simulink model "inclass1006"  (R2026a)
settings: Solver=FixedStepAuto  StopTime=inf  FixedStep=0.05
libraries: robotlib x9
settings Model: Creator=sprinkle  LastModifiedBy=sprinkle
settings HardwareCC: ProdHWDeviceType=Generic->Unspecified (assume 32-bit Generic)
settings RTWCC: SystemTargetFile=ert.tlc  HardwareBoard=Robot Operating System (ROS)  TLCOptions="-aInlineSetEventsForThisBaseRateFcn=TLC_FALSE -aSuppressMultiTaskScheduler=TLC_FALSE  -aRateBasedStepFcn=0"  GenCodeOnly=on  Toolchain=Catkin  TargetLang=C++  Description=Embedded Coder

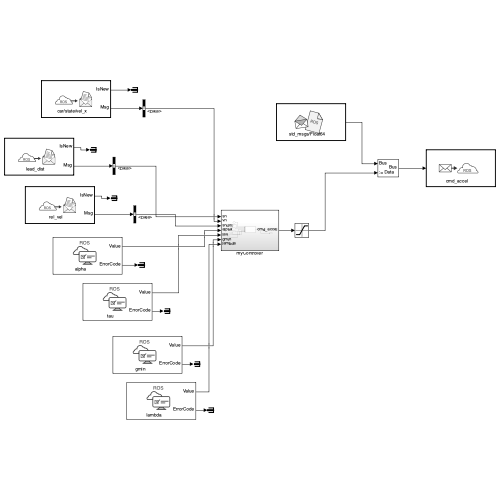
[thumbnail: Simulink's stored preview of the top-level diagram]
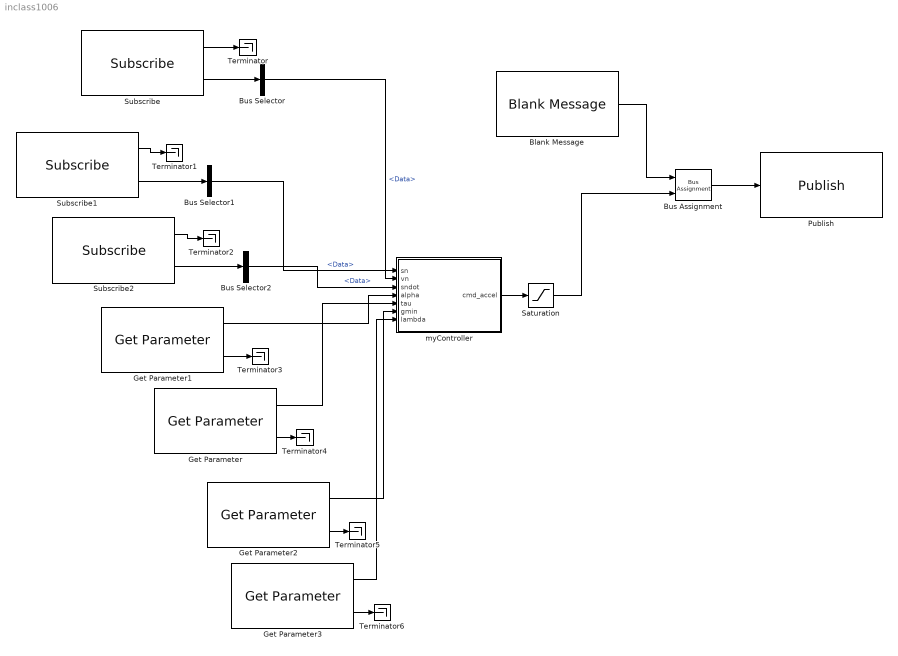
== system inclass1006 ==
  Blank Message : robotlib/Blank Message  messageClass=Message  entityType=std_msgs/Float64  messageType=std_msgs/Float64  SampleTime=inf  legacyBusStruct=off
  Bus Assignment : BusAssignment  AssignedSignals=Data
  Bus Selector : BusSelector  OutputSignals=Data
  Bus Selector1 : BusSelector  OutputSignals=Data
  Bus Selector2 : BusSelector  OutputSignals=Data
  Get Parameter : robotlib/Get Parameter  ParameterSource=Specify your own  ParameterName=tau  ParameterType=double  ParameterMaxArrayLength=16  ParameterInitialValue=2.0  SampleTime=-1  ShowErrorCodeOutput=on  ModelName=inclass1006  BlockId=ParamGet_inclass1006_18
  Get Parameter1 : robotlib/Get Parameter  ParameterSource=Specify your own  ParameterName=alpha  ParameterType=double  ParameterMaxArrayLength=16  ParameterInitialValue=1.1  SampleTime=-1  ShowErrorCodeOutput=on  ModelName=inclass1006  BlockId=ParamGet_inclass1006_19
  Get Parameter2 : robotlib/Get Parameter  ParameterSource=Specify your own  ParameterName=gmin  ParameterType=double  ParameterMaxArrayLength=16  ParameterInitialValue=3  SampleTime=-1  ShowErrorCodeOutput=on  ModelName=inclass1006  BlockId=ParamGet_inclass1006_52
  Get Parameter3 : robotlib/Get Parameter  ParameterSource=Specify your own  ParameterName=lambda  ParameterType=double  ParameterMaxArrayLength=16  ParameterInitialValue=0.1  SampleTime=-1  ShowErrorCodeOutput=on  ModelName=inclass1006  BlockId=ParamGet_inclass1006_52
  Publish : robotlib/Publish  topicSource=Specify your own  topic=cmd_accel  messageType=std_msgs/Float64  legacyBusStruct=off  messageQueueLength=1
  Saturation : Saturate  UpperLimit=1.5  LowerLimit=-3.0
  Subscribe : robotlib/Subscribe  topicSource=Specify your own  topic=car/state/vel_x  messageType=std_msgs/Float64  SampleTime=-1  legacyBusStruct=off  messageQueueLength=1
  Subscribe1 : robotlib/Subscribe  topicSource=Specify your own  topic=lead_dist  messageType=std_msgs/Float64  SampleTime=-1  legacyBusStruct=off  messageQueueLength=1
  Subscribe2 : robotlib/Subscribe  topicSource=Specify your own  topic=rel_vel  messageType=std_msgs/Float64  SampleTime=-1  legacyBusStruct=off  messageQueueLength=1
  Terminator{,1..6} (7 alike) : Terminator
  myController : Subsystem
  wires:
  Subscribe/2 -> Bus Selector/1
  Subscribe/1 -> Terminator/1
  Subscribe1/1 -> Terminator1/1
  Blank Message/1 -> Bus Assignment/1
  Bus Assignment/1 -> Publish/1
  Bus Selector/1 -> myController/2(vn)  "<Data>"
  myController/1(cmd_accel) -> Saturation/1
  Get Parameter/1 -> myController/5(tau)
  Get Parameter1/1 -> myController/4(alpha)
  Saturation/1 -> Bus Assignment/2
  Subscribe1/2 -> Bus Selector1/1
  Bus Selector1/1 -> myController/1(sn)  "<Data>"
  Subscribe2/1 -> Terminator2/1
  Bus Selector2/1 -> myController/3(sndot)  "<Data>"
  Subscribe2/2 -> Bus Selector2/1
  Get Parameter1/2 -> Terminator3/1
  Get Parameter/2 -> Terminator4/1
  Get Parameter2/2 -> Terminator5/1
  Get Parameter3/2 -> Terminator6/1
  Get Parameter2/1 -> myController/6(gmin)
  Get Parameter3/1 -> myController/7(lambda)

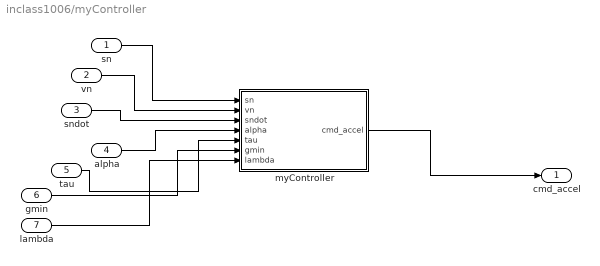
== system inclass1006/myController ==
  sn : Inport
  vn : Inport  Port=2
  sndot : Inport  Port=3
  alpha : Inport  Port=4
  tau : Inport  Port=5
  gmin : Inport  Port=6
  lambda : Inport  Port=7
  myController : Subsystem
  cmd_accel : Outport
  wires:
  myController/1(cmd_accel) -> cmd_accel/1
  tau/1 -> myController/5(tau)
  alpha/1 -> myController/4(alpha)
  sn/1 -> myController/1(sn)
  vn/1 -> myController/2(vn)
  sndot/1 -> myController/3(sndot)
  gmin/1 -> myController/6(gmin)
  lambda/1 -> myController/7(lambda)

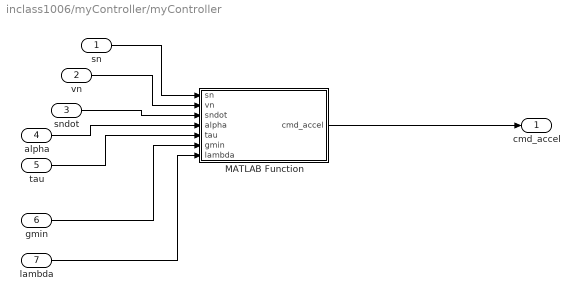
== system inclass1006/myController/myController ==
  sn : Inport
  vn : Inport  Port=2
  sndot : Inport  Port=3
  alpha : Inport  Port=4
  tau : Inport  Port=5
  gmin : Inport  Port=6
  lambda : Inport  Port=7
  MATLAB Function : MATLAB Function  TreatAsAtomicUnit=on
  cmd_accel : Outport
  wires:
  MATLAB Function/1(cmd_accel) -> cmd_accel/1
  tau/1 -> MATLAB Function/5(tau)
  alpha/1 -> MATLAB Function/4(alpha)
  sn/1 -> MATLAB Function/1(sn)
  vn/1 -> MATLAB Function/2(vn)
  sndot/1 -> MATLAB Function/3(sndot)
  gmin/1 -> MATLAB Function/6(gmin)
  lambda/1 -> MATLAB Function/7(lambda)

== matlab function inclass1006/myController/myController/MATLAB Function ==
  data: sn input; cmd_accel output; vn input; sndot input; alpha input; tau input; gmin input; lambda input
function cmd_accel = fcn(sn,vn,sndot,alpha,tau,gmin,lambda)
                    
cmd_accel = alpha * (sn - tau*vn - gmin) + lambda*sndot;
